simulink model "ps_25V_12kA_r"  (R2026b)
settings: Solver=ode23tb  StopTime=param.sim.simlength  FixedStep=param.glb_time.tc  MaxStep=param.glb_time.tc
values from neighbouring files (symbols this model uses):
  param = struct()    [init_model.m]
undefined symbols (not defined in the file or in its folder): magnitude
libraries: fl_lib x106, nesl_utility x71, afe_uvw_ctrl x5, ee_legacy_lib x5, discrete_time_low_pass_filter x2, three_windings_transformer x2, pi_ctrl x2, threephase_inductor_lib x1, dclink_for_two_levels x1, three_phase_pwm_modulator x1, three_phase_inverter_ideal_switch_based_model x1, three_phase_inverter_igbt_advanced_thermal_model x1
(part 3 of 5)

== system ps_25V_12kA_r/full_bridge_converter/phase_shift_full_bridge_ctrl/ui_ctrl ==
  i_pu_dab_input : Inport
  u_pu_dab_output : Inport  Port=2
  i_pu_dab_output_ref : Inport  Port=3
  i_ac_pu_1 : Inport  Port=4
  Trigger : TriggerPort  VariantControl=(inherit)  PortDimensions=1
  Goto Tag Visibility : GotoTagVisibility  GotoTag=idc_trafo_2
  Goto Tag Visibility1 : GotoTagVisibility  GotoTag=idc_trafo_1
  Goto Tag Visibility2 : GotoTagVisibility  GotoTag=idc_trafo_2_comp
  Goto Tag Visibility3 : GotoTagVisibility  GotoTag=idc_trafo_1_comp
  Goto Tag Visibility4 : GotoTagVisibility  GotoTag=i_pu_psfbc_output_ref
  Goto Tag Visibility5 : GotoTagVisibility  GotoTag=uout_pu_psfbc
  Goto Tag Visibility6 : GotoTagVisibility  GotoTag=i_ctrl_out_psfbc
  Goto Tag Visibility7 : GotoTagVisibility  GotoTag=i_pu_psfbc_output
  d1_m : Subsystem
  dc_trafo_current_measurements_and_compensation : Subsystem
  psfbc_ctrl : Subsystem
  scopes : Subsystem
  d1m : Outport
  phase_displacement : Outport  Port=2
  wires:
  i_pu_dab_input/1 -> psfbc_ctrl/1(i_pu_psfbc_output)
  u_pu_dab_output/1 -> psfbc_ctrl/2(u_pu_psfbc_output)
  i_pu_dab_output_ref/1 -> psfbc_ctrl/3(i_pu_psfbc_output_ref)
  psfbc_ctrl/1(phase_displacement) -> phase_displacement/1
  i_ac_pu_1/1 -> dc_trafo_current_measurements_and_compensation/1(i_ac_pu_1)
  d1_m/1(d1m) -> d1m/1

== system ps_25V_12kA_r/grid/grid_emulator/3ph_Dyg_ssc ==
  Electrical Reference1 : fl_lib/Electrical/Electrical Elements/Electrical Reference
  PS Terminator : fl_lib/Physical Signals/Sinks/PS Terminator
  PS Terminator1 : fl_lib/Physical Signals/Sinks/PS Terminator
  PS Terminator2 : fl_lib/Physical Signals/Sinks/PS Terminator
  configurable_trafo : SimscapeComponentBlock  Description=Configurable transformer: one or two three-phase primaries (star or delta), secondary three-phase (star or delta, any clock number) or single-phase (turns distribution ws) on a three-limb core. Component configurable_transformer.configurable_transformer (pwr-control/library, foundation/electrical_machines/+configurable_transformer).  SourceFile=configurable_transformer.configurable_transformer  ComponentPath=configurable_transformer.configurable_transformer  ComponentVariants="[\"configurable_transformer.configurable_transformer\"]"  ComponentVariantNames="[\"configurable_transformer\"]"  ClassName=configurable_transformer  SchemaVersion=1  primaries=configurable_transformer.n_primaries.one  conn1=configurable_transformer.connection.delta  conn2=configurable_transformer.connection.star  clock2=0  secondary=configurable_transformer.secondary_winding.star  clock3=param.grid.emu.trafo.pu.clock3  ws=[1, -1, 0]  Sr=param.grid.emu.trafo.pwr_nom A*V  V1=param.grid.emu.trafo.u1_nom V  V2=400 V  V3=param.grid.emu.trafo.u2_nom V  fr=param.grid.emu.trafo.f_nom Hz  r1=param.grid.emu.trafo.pu.r1  l1=param.grid.emu.trafo.pu.l1  r2=0.005  l2=0.030  r3=param.grid.emu.trafo.pu.r3  l3=param.grid.emu.trafo.pu.l3  lm=param.grid.emu.trafo.pu.lm  lm0=param.grid.emu.trafo.pu.lm0  rfe=param.grid.emu.trafo.pu.rfe  i1a_specify=off  i1a_priority=None  i1a=0 A  i1a_nominal_specify=off  i1a_nominal_value=1  i1a_nominal_unit=A  i1b_specify=off  i1b_priority=None  i1b=0 A  i1b_nominal_specify=off  i1b_nominal_value=1  i1b_nominal_unit=A  i1c_specify=off  i1c_priority=None  i1c=0 A  i1c_nominal_specify=off  i1c_nominal_value=1  i1c_nominal_unit=A  i2a_specify=off  i2a_priority=None  i2a=0 A  i2a_nominal_specify=off  i2a_nominal_value=1  i2a_nominal_unit=A  i2b_specify=off  i2b_priority=None  i2b=0 A  i2b_nominal_specify=off  i2b_nominal_value=1  i2b_nominal_unit=A  i2c_specify=off  i2c_priority=None  i2c=0 A  i2c_nominal_specify=off  i2c_nominal_value=1  i2c_nominal_unit=A  i3a_specify=off  i3a_priority=None  i3a=0 A  i3a_nominal_specify=off  i3a_nominal_value=1  i3a_nominal_unit=A  i3b_specify=off  i3b_priority=None  i3b=0 A  i3b_nominal_specify=off  i3b_nominal_value=1  i3b_nominal_unit=A  i3c_specify=off  i3c_priority=None  i3c=0 A  i3c_nominal_specify=off  i3c_nominal_value=1  i3c_nominal_unit=A  i3_specify=off  i3_priority=None  i3=0 A  i3_nominal_specify=off  i3_nominal_value=1  i3_nominal_unit=A
      settings: CopyFcn=simscape.sscblock.internal.componentBlockCallback(gcbh,'COPY')  PreCopyFcn=simscape.sscblock.internal.componentBlockCallback(gcbh,'PRECOPY')  PreDeleteFcn=simscape.sscblock.internal.componentBlockCallback(gcbh,'PREDELETE')
      mask Type: Configurable Transformer
  ua : PMIOPort  Side=Right
  ub : PMIOPort  Port=2  Side=Right
  uc : PMIOPort  Port=3  Side=Right
  Ua : PMIOPort  Port=4  Side=Left
  Ub : PMIOPort  Port=5  Side=Left
  Uc : PMIOPort  Port=6  Side=Left
  connections:
  Uc/RConn1 -- configurable_trafo/LConn3
  configurable_trafo/LConn2 -- Ub/RConn1
  configurable_trafo/RConn1 -- ua/RConn1
  configurable_trafo/LConn1 -- Ua/RConn1
  ub/RConn1 -- configurable_trafo/RConn2
  configurable_trafo/RConn3 -- uc/RConn1
  Electrical Reference1/LConn1 -- configurable_trafo/RConn4
  PS Terminator/LConn1 -- configurable_trafo/RConn5
  PS Terminator1/LConn1 -- configurable_trafo/RConn6
  configurable_trafo/RConn7 -- PS Terminator2/LConn1

== system ps_25V_12kA_r/grid/grid_emulator/threephase_vi_measures ==
  Bus Creator : BusCreator  Inputs=6
  Current Sensor : fl_lib/Electrical/Electrical Sensors/Current Sensor
  Current Sensor1 : fl_lib/Electrical/Electrical Sensors/Current Sensor
  Current Sensor2 : fl_lib/Electrical/Electrical Sensors/Current Sensor
  Electrical Reference1 : fl_lib/Electrical/Electrical Elements/Electrical Reference
  Voltage Sensor : fl_lib/Electrical/Electrical Sensors/Voltage Sensor
  Voltage Sensor1 : fl_lib/Electrical/Electrical Sensors/Voltage Sensor
  Voltage Sensor2 : fl_lib/Electrical/Electrical Sensors/Voltage Sensor
  i : Selector  InputPortWidth=6  IndexOptions=Index vector (dialog)  Indices=[4 5 6]  OutputSizes=1  RuntimeRangeChecks=off
  ia_grid : nesl_utility/PS-Simulink Converter  PhysicalDomain=network_engine_domain  SubClassName=ps_output  LeftPortType=input  RightPortType=output  PseudoPeriodic=off  Frequencies=[]  VectorFormat=1-D array  Unit=A  AffineConversion=off
  ib_grid : nesl_utility/PS-Simulink Converter  PhysicalDomain=network_engine_domain  SubClassName=ps_output  LeftPortType=input  RightPortType=output  PseudoPeriodic=off  Frequencies=[]  VectorFormat=1-D array  Unit=A  AffineConversion=off
  ic_grid : nesl_utility/PS-Simulink Converter  PhysicalDomain=network_engine_domain  SubClassName=ps_output  LeftPortType=input  RightPortType=output  PseudoPeriodic=off  Frequencies=[]  VectorFormat=1-D array  Unit=A  AffineConversion=off
  u : Selector  InputPortWidth=6  IndexOptions=Index vector (dialog)  Indices=[1 2 3]  OutputSizes=1  RuntimeRangeChecks=off
  ua_grid : nesl_utility/PS-Simulink Converter  PhysicalDomain=network_engine_domain  SubClassName=ps_output  LeftPortType=input  RightPortType=output  PseudoPeriodic=off  Frequencies=[]  VectorFormat=1-D array  Unit=V  AffineConversion=off
  ub_grid : nesl_utility/PS-Simulink Converter  PhysicalDomain=network_engine_domain  SubClassName=ps_output  LeftPortType=input  RightPortType=output  PseudoPeriodic=off  Frequencies=[]  VectorFormat=1-D array  Unit=V  AffineConversion=off
  uc_grid : nesl_utility/PS-Simulink Converter  PhysicalDomain=network_engine_domain  SubClassName=ps_output  LeftPortType=input  RightPortType=output  PseudoPeriodic=off  Frequencies=[]  VectorFormat=1-D array  Unit=V  AffineConversion=off
  Ua : PMIOPort  Side=Left
  ua : PMIOPort  Port=2  Side=Right
  Ub : PMIOPort  Port=3  Side=Left
  ub : PMIOPort  Port=4  Side=Right
  Uc : PMIOPort  Port=5  Side=Left
  uc : PMIOPort  Port=6  Side=Right
  tag scope: i_abc_line=global, u_abc_line=global
  wires:
  Bus Creator/1 -> i/1, u/1  "vi_data"
  ib_grid/1 -> Bus Creator/5  "ib"
  ia_grid/1 -> Bus Creator/4  "ia"
  ic_grid/1 -> Bus Creator/6  "ic"
  ua_grid/1 -> Bus Creator/1  "ua"
  ub_grid/1 -> Bus Creator/2  "ub"
  uc_grid/1 -> Bus Creator/3  "uc"
  i/1 -> [i_abc_line]
  u/1 -> [u_abc_line]
  connections:
  Current Sensor1/LConn1 -- Ub/RConn1 -- Voltage Sensor1/LConn1
  Electrical Reference1/LConn1 -- Voltage Sensor/RConn2 -- Voltage Sensor2/RConn2 -- Voltage Sensor1/RConn2
  Voltage Sensor/RConn1 -- ua_grid/LConn1
  Current Sensor/RConn2 -- ua/RConn1
  Voltage Sensor1/RConn1 -- ub_grid/LConn1
  Voltage Sensor2/LConn1 -- Current Sensor2/LConn1 -- Uc/RConn1
  Current Sensor/LConn1 -- Ua/RConn1 -- Voltage Sensor/LConn1
  Current Sensor1/RConn2 -- ub/RConn1
  Voltage Sensor2/RConn1 -- uc_grid/LConn1
  ib_grid/LConn1 -- Current Sensor1/RConn1
  ia_grid/LConn1 -- Current Sensor/RConn1
  ic_grid/LConn1 -- Current Sensor2/RConn1
  Current Sensor2/RConn2 -- uc/RConn1

== system ps_25V_12kA_r/afe_abc_mod1/AFE_control/afe_control/FRT-VDE4110 ==
  Constant4 : Constant  Value=0
  Mux : Mux
  Mux1 : Mux  Inputs=2
  enable : Step  Time=param.frt.data.settle_time  FinalValue=param.frt.data.enable_frt_1 + param.frt.data.enable_frt_2
  frt_detection_output : Scope  NumInputPorts=3
      settings: ActiveDisplayYMinimum=-0.12499999999999997  ActiveDisplayYMaximum=1.125
  frt_vde4110 : afe_uvw_ctrl/frt_vde4110  p=param.afe.uvw
  positive_reactive_current_reference : Subsystem
  reset : Step  Time=0.025  InitialValue=1  FinalValue=0
  tag scope: frt_active=scoped, i_grid_seq_ref=scoped, pwr_lim_enable=scoped
  wires:
  frt_vde4110/2 -> [frt_active], frt_detection_output/2  "frt_active"
  frt_vde4110/3 -> [pwr_lim_enable], frt_detection_output/3  "pwr_lim_enable"
  frt_vde4110/4 -> frt_detection_output/1  "frt_state"
  reset/1 -> frt_vde4110/4  "reset"
  enable/1 -> frt_vde4110/3  "enable"
  [v_grid_neg_eta_avg] -> Mux/4
  [v_grid_neg_xi_avg] -> Mux/3
  [v_grid_pos_eta_avg] -> Mux/2
  [v_grid_pos_xi_avg] -> Mux/1
  Mux/1 -> frt_vde4110/1
  positive_reactive_current_reference/1(i_react_pos_ref) -> [i_react_pos_ref]
  Constant4/1 -> [i_react_neg_ref]
  frt_vde4110/1 -> [i_grid_seq_ref]
  [i_react_neg_ref] -> Mux1/2
  [i_react_pos_ref] -> Mux1/1
  Mux1/1 -> frt_vde4110/2

== system ps_25V_12kA_r/afe_abc_mod1/AFE_control/afe_control/current_ctrl ==
  i_xi_ref : Inport
  Mux : Mux  Inputs=3
  current_ctrl_uvw : afe_uvw_ctrl/current_ctrl_uvw  p=param.afe.uvw
  isa_ref/isa : Scope  NumInputPorts=2
      settings: ActiveDisplayYMinimum=-3.5647345146351177  ActiveDisplayYMaximum=2.2290599372806974
  u_alpha_beta_gamma_out : Outport
  wires:
  i_xi_ref/1 -> current_ctrl_uvw/1  "is_pos_xi_ref"
  [i_stack_neg_xi_ref] -> Mux/2  "is_neg_xi_ref"
  [i_stack_pos_eta_ref] -> Mux/1  "is_pos_eta_ref"
  [i_stack_neg_eta_ref] -> Mux/3  "is_neg_eta_ref"
  [phase_grid_pll] -> current_ctrl_uvw/4
  [isd_abc_pu] -> current_ctrl_uvw/3
  current_ctrl_uvw/1 -> u_alpha_beta_gamma_out/1
  current_ctrl_uvw/2 -> isa_ref/isa/1
  current_ctrl_uvw/3 -> isa_ref/isa/2
  Mux/1 -> current_ctrl_uvw/2

== system ps_25V_12kA_r/afe_abc_mod1/AFE_control/afe_control/data_to_worspace_module_1 ==
  Bus Creator : BusCreator  Inputs=5
  dq_pll : Subsystem
  inner_current_tracking : Subsystem
  pwr_meter : Subsystem
  sequences_data : Subsystem
  m : Outport
  wires:
  Bus Creator/1 -> m/1
  sequences_data/1(m_seq) -> Bus Creator/1  "sequences_data"
  pwr_meter/1(m_pwr_meter) -> Bus Creator/2  "pwr_meter"
  inner_current_tracking/1(m_inner_current_tracking) -> Bus Creator/3  "m_inner_current_tracking"
  [local_time] -> Bus Creator/5  "local_time"
  dq_pll/1(dqPLLs) -> Bus Creator/4  "dq_pll"

== system ps_25V_12kA_r/afe_abc_mod1/AFE_control/afe_control/grid_current_sequences_and_reactive_pwr_ctrl ==
  ig_abc_pu : Inport
  Abs : Abs  SaturateOnIntegerOverflow=off
  Demux : Demux  Outputs=3
  Demux1 : Demux
  Saturation : Saturate  UpperLimit=2  LowerLimit=0.1
  Terminator : Terminator
  grid_current_sequences_q_ctrl : afe_uvw_ctrl/grid_current_sequences_q_ctrl  p=param.afe.uvw
  tag scope: i_grid_neg_eta_avg=scoped, i_grid_neg_xi_avg=scoped, i_grid_pos_eta_avg=scoped, i_grid_pos_xi_avg=scoped, i_stack_neg_eta_ref=scoped, i_stack_neg_xi_ref=scoped, i_stack_pos_eta_ref=scoped
  wires:
  [phase_grid_pll] -> grid_current_sequences_q_ctrl/2
  ig_abc_pu/1 -> grid_current_sequences_q_ctrl/1
  grid_current_sequences_q_ctrl/1 -> Demux/1
  Demux/1 -> [i_stack_pos_eta_ref]
  grid_current_sequences_q_ctrl/2 -> Demux1/1
  Demux1/1 -> [i_grid_pos_xi_avg]
  Demux1/2 -> [i_grid_pos_eta_avg]
  Demux1/3 -> [i_grid_neg_xi_avg]
  Demux1/4 -> [i_grid_neg_eta_avg]
  grid_current_sequences_q_ctrl/3 -> Terminator/1
  [i_grid_seq_ref] -> grid_current_sequences_q_ctrl/4
  Saturation/1 -> grid_current_sequences_q_ctrl/3
  [omega_grid_pll_pu] -> Abs/1
  Abs/1 -> Saturation/1
  Demux/2 -> [i_stack_neg_xi_ref]
  Demux/3 -> [i_stack_neg_eta_ref]

== system ps_25V_12kA_r/afe_abc_mod1/AFE_control/afe_control/grid_phase_acquisition ==
  grid_phase : Inport
  Quantizer : Quantizer  QuantizationInterval=param.meas.adc_quantization
  Unit Delay : UnitDelay  SampleTime=-1
  Zero-Order Hold : ZeroOrderHold  SampleTime=-1
  grid_phased : Outport
  wires:
  Zero-Order Hold/1 -> Quantizer/1
  Unit Delay/1 -> grid_phased/1
  grid_phase/1 -> Zero-Order Hold/1
  Quantizer/1 -> Unit Delay/1

== system ps_25V_12kA_r/afe_abc_mod1/AFE_control/afe_control/grid_voltage_phase_lock_loops ==
  ug_abc_pu : Inport
  Bus Creator2 : BusCreator  Inputs=2
  FHT-PLL performance : Scope  NumInputPorts=2
      settings: ActiveDisplayYMinimum=-1.32501220703125  ActiveDisplayYMaximum=1.30987548828125  DataLoggingVariableName=ScopeData8
  FHT-PLL_simulink : Subsystem
  tag scope: omega_grid_pll_pu=scoped, phase_grid_pll=scoped
  wires:
  FHT-PLL_simulink/1(gamma_grid_fht_pll) -> [phase_grid_pll]
  FHT-PLL_simulink/2(omega_grid_fht_pll) -> [omega_grid_pll_pu]
  ug_abc_pu/1 -> FHT-PLL performance/1, FHT-PLL_simulink/1(ug_abc_pu)
  Bus Creator2/1 -> FHT-PLL performance/2
  [omega_grid_pll_pu] -> Bus Creator2/2  "omega_grid_fht_pll"
  [phase_grid_pll] -> Bus Creator2/1  "phase_grid_fht_pll"

== system ps_25V_12kA_r/afe_abc_mod1/AFE_control/afe_control/grid_voltage_sequences ==
  Abs : Abs  SaturateOnIntegerOverflow=off
  Demux : Demux
  Demux1 : Demux  Outputs=2
  Saturation : Saturate  UpperLimit=2  LowerLimit=0.1
  Terminator : Terminator
  grid_voltage_sequences1 : afe_uvw_ctrl/grid_voltage_sequences  p=param.afe.uvw
  tag scope: ug_alpha_pu=scoped, ug_beta_pu=scoped, v_grid_neg_eta_avg=scoped, v_grid_neg_xi_avg=scoped, v_grid_pos_eta_avg=scoped, v_grid_pos_xi_avg=scoped
  wires:
  [ugd_abc_pu] -> grid_voltage_sequences1/1
  [phase_grid_pll] -> grid_voltage_sequences1/2
  Abs/1 -> Saturation/1
  [omega_grid_pll_pu] -> Abs/1
  Saturation/1 -> grid_voltage_sequences1/3
  grid_voltage_sequences1/1 -> Demux/1
  Demux/4 -> [v_grid_neg_eta_avg]
  Demux/3 -> [v_grid_neg_xi_avg]
  Demux/2 -> [v_grid_pos_eta_avg]
  Demux/1 -> [v_grid_pos_xi_avg]
  grid_voltage_sequences1/3 -> Demux1/1
  Demux1/1 -> [ug_alpha_pu]
  Demux1/2 -> [ug_beta_pu]
  grid_voltage_sequences1/2 -> Terminator/1

== system ps_25V_12kA_r/afe_abc_mod1/AFE_control/afe_control/ig afe quantizzation and one step delay ==
  ig_abc_pu : Inport
  Demux1 : Demux  Outputs=3
  Mux1 : Mux  Inputs=3
  ig afe quantizzation and one step delay : Subsystem
  igd_abc_pu : Outport
  wires:
  Demux1/1 -> ig afe quantizzation and one step delay/1(ig_u_pu)
  Demux1/2 -> ig afe quantizzation and one step delay/2(ig_v_pu)
  ig_abc_pu/1 -> Demux1/1
  Mux1/1 -> igd_abc_pu/1
  Demux1/3 -> ig afe quantizzation and one step delay/3(ig_w_pu)
  ig afe quantizzation and one step delay/2(igd_v_pu) -> Mux1/2
  ig afe quantizzation and one step delay/1(igd_u_pu) -> Mux1/1
  ig afe quantizzation and one step delay/3(igd_w_pu) -> Mux1/3

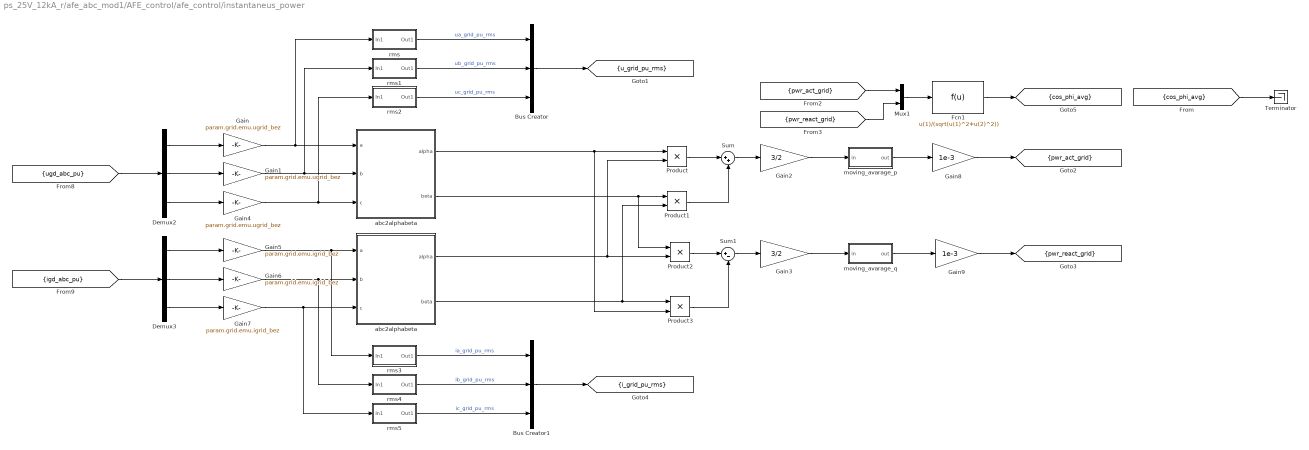
== system ps_25V_12kA_r/afe_abc_mod1/AFE_control/afe_control/instantaneus_power ==
  Bus Creator : BusCreator  Inputs=3
  Bus Creator1 : BusCreator  Inputs=3
  Demux2 : Demux  Outputs=3
  Demux3 : Demux  Outputs=3
  Fcn1 : Fcn  Expr=u(1)/(sqrt(u(1)^2+u(2)^2))
  Gain : Gain  Gain=param.grid.emu.ugrid_bez
  Gain1 : Gain  Gain=param.grid.emu.ugrid_bez
  Gain2 : Gain  Gain=3/2
  Gain3 : Gain  Gain=3/2
  Gain4 : Gain  Gain=param.grid.emu.ugrid_bez
  Gain5 : Gain  Gain=param.grid.emu.igrid_bez
  Gain6 : Gain  Gain=param.grid.emu.igrid_bez
  Gain7 : Gain  Gain=param.grid.emu.igrid_bez
  Gain8 : Gain  Gain=1e-3
  Gain9 : Gain  Gain=1e-3
  Mux1 : Mux  Inputs=2
  Product{,1..3} (4 alike) : Product  RndMeth=Zero
  Sum : Sum  Inputs=|++
  Sum1 : Sum  Inputs=|+-
  Terminator : Terminator
  abc2alphabeta : Subsystem
  "abc2alphabeta " : Subsystem
  moving_avarage_p : Subsystem
  moving_avarage_q : Subsystem
  rms : Subsystem
  rms1 : Subsystem
  rms2 : Subsystem
  rms3 : Subsystem
  rms4 : Subsystem
  rms5 : Subsystem
  tag scope: cos_phi_avg=scoped, i_grid_pu_rms=scoped, pwr_act_grid=scoped, pwr_react_grid=scoped, u_grid_pu_rms=scoped
  wires:
  abc2alphabeta/2("beta ") -> Product1/1, Product2/1
  "abc2alphabeta "/2("beta ") -> Product1/2, Product3/1
  abc2alphabeta/1("alpha ") -> Product3/2, Product/1
  "abc2alphabeta "/1("alpha ") -> Product2/2, Product/2
  Product/1 -> Sum/1
  Product1/1 -> Sum/2
  Product2/1 -> Sum1/1
  Product3/1 -> Sum1/2
  Sum1/1 -> Gain3/1
  Sum/1 -> Gain2/1
  Gain2/1 -> moving_avarage_p/1(in)
  Gain3/1 -> moving_avarage_q/1(in)
  [pwr_react_grid] -> Mux1/2
  Mux1/1 -> Fcn1/1
  Fcn1/1 -> [cos_phi_avg]
  [pwr_act_grid] -> Mux1/1
  rms/1(Out1) -> Bus Creator/1  "ua_grid_pu_rms"
  rms2/1(Out1) -> Bus Creator/3  "uc_grid_pu_rms"
  rms1/1(Out1) -> Bus Creator/2  "ub_grid_pu_rms"
  moving_avarage_p/1(out) -> Gain8/1
  moving_avarage_q/1(out) -> Gain9/1
  Demux2/1 -> Gain/1
  Demux2/2 -> Gain1/1
  Demux2/3 -> Gain4/1
  Demux3/1 -> Gain5/1
  Demux3/2 -> Gain6/1
  Demux3/3 -> Gain7/1
  Gain/1 -> rms/1(In1), abc2alphabeta/1(a)
  Gain1/1 -> rms1/1(In1), abc2alphabeta/2(b)
  Gain4/1 -> rms2/1(In1), abc2alphabeta/3(c)
  Gain5/1 -> rms3/1(In1), "abc2alphabeta "/1(a)
  Gain6/1 -> rms4/1(In1), "abc2alphabeta "/2(b)
  Gain7/1 -> rms5/1(In1), "abc2alphabeta "/3(c)
  Gain8/1 -> [pwr_act_grid]
  Gain9/1 -> [pwr_react_grid]
  [ugd_abc_pu] -> Demux2/1
  [igd_abc_pu] -> Demux3/1
  Bus Creator/1 -> [u_grid_pu_rms]
  rms4/1(Out1) -> Bus Creator1/2  "ib_grid_pu_rms"
  rms3/1(Out1) -> Bus Creator1/1  "ia_grid_pu_rms"
  rms5/1(Out1) -> Bus Creator1/3  "ic_grid_pu_rms"
  Bus Creator1/1 -> [i_grid_pu_rms]
  [cos_phi_avg] -> Terminator/1

== system ps_25V_12kA_r/afe_abc_mod1/AFE_control/afe_control/interesting scopes ==
  current_sequences_mod1 : Scope  NumInputPorts=4
      settings: ActiveDisplayYMinimum=-0.97178065031766891  ActiveDisplayYMaximum=1.9392475411295891  DataLoggingVariableName=ScopeData2
  i_grid_seq_ref : Scope
      settings: ActiveDisplayYMinimum=-1.1499999999999995  ActiveDisplayYMaximum=0.34999999999999981
  voltage_sequences_mod1 : Scope  NumInputPorts=4
      settings: ActiveDisplayYMinimum=-1.2405151816982258  ActiveDisplayYMaximum=1.2605257614333911
  wires:
  [v_grid_neg_eta_avg] -> voltage_sequences_mod1/4  "u_grid_neg_eta"
  [i_grid_neg_xi_avg] -> current_sequences_mod1/3  "i_grid_neg_xi"
  [v_grid_pos_eta_avg] -> voltage_sequences_mod1/2  "u_grid_pos_eta"
  [v_grid_neg_xi_avg] -> voltage_sequences_mod1/3  "u_grid_neg_xi"
  [i_grid_pos_xi_avg] -> current_sequences_mod1/1  "i_grid_pos_xi"
  [i_grid_neg_eta_avg] -> current_sequences_mod1/4  "i_grid_neg_eta"
  [v_grid_pos_xi_avg] -> voltage_sequences_mod1/1  "u_grid_pos_xi"
  [i_grid_pos_eta_avg] -> current_sequences_mod1/2  "i_grid_pos_eta"
  [i_grid_seq_ref] -> i_grid_seq_ref/1  "i_grid_seq_ref"

== system ps_25V_12kA_r/afe_abc_mod1/AFE_control/afe_control/is afe quantizzation and one step delay ==
  is_abc_pu : Inport
  Demux : Demux  Outputs=3
  Mux : Mux  Inputs=3
  is afe quantizzation and one step delay : Subsystem
  isd_abc_pu : Outport
  wires:
  is afe quantizzation and one step delay/2(isd_v_pu) -> Mux/2
  is_abc_pu/1 -> Demux/1
  is afe quantizzation and one step delay/3(isd_w_pu) -> Mux/3
  is afe quantizzation and one step delay/1(isd_u_pu) -> Mux/1
  Demux/1 -> is afe quantizzation and one step delay/1(is_u_pu)
  Mux/1 -> isd_abc_pu/1
  Demux/3 -> is afe quantizzation and one step delay/3(is_w_pu)
  Demux/2 -> is afe quantizzation and one step delay/2(is_v_pu)

== system ps_25V_12kA_r/afe_abc_mod1/AFE_control/afe_control/islanding_mode_detector ==
  gamma : Inport
  alpha : Inport  Port=2
  beta : Inport  Port=3
  Constant : Constant
  Mux : Mux  Inputs=2
  island_detection : Scope  NumInputPorts=3
      settings: ActiveDisplayYMinimum=-13.028939727220205  ActiveDisplayYMaximum=117.26045754498188  DataLoggingVariableName=ScopeData10
  islanding_detector : afe_uvw_ctrl/islanding_detector  p=param.afe.uvw
  wires:
  Mux/1 -> islanding_detector/1
  alpha/1 -> Mux/1  "u_grid_alpha"
  beta/1 -> Mux/2  "u_grid_beta"
  gamma/1 -> islanding_detector/2  "gamma_grid"
  [omega_grid_pll_pu] -> islanding_detector/3
  Constant/1 -> islanding_detector/4
  islanding_detector/1 -> island_detection/1
  islanding_detector/2 -> island_detection/2
  islanding_detector/3 -> island_detection/3

== system ps_25V_12kA_r/afe_abc_mod1/AFE_control/afe_control/phase_compensation_1 ==
  local_time : Inport
  master_time : Inport  Port=2
  Zero-Order Hold : ZeroOrderHold  SampleTime=-1
  Zero-Order Hold1 : ZeroOrderHold  SampleTime=-1
  alignment_eval_afe1 : Subsystem
  y : Outport
  wires:
  local_time/1 -> Zero-Order Hold/1
  master_time/1 -> Zero-Order Hold1/1
  alignment_eval_afe1/1(dp) -> y/1
  Zero-Order Hold/1 -> alignment_eval_afe1/1(local_time)
  Zero-Order Hold1/1 -> alignment_eval_afe1/2(master_time)

== system ps_25V_12kA_r/afe_abc_mod1/AFE_control/afe_control/space_vector ==
  uab_out : Inport
  Bus Creator : BusCreator  Inputs=3
  Bus Selector : BusSelector  OutputSignals=da,db,dc
  C Caller : CCaller  FunctionName=sv_pwm_cm_process_simulink  PortSpecificationStruct="%)30     .    B H   8    (     @         %    \"     8    !     0         %  0 \"0    $    _    07)G3F%M90  4&]R=$YA;64 4V-O<&4     26YD97@     5'EP90      4VEZ90      27-';&]B86P   X    P    !@    @    $          4    (     0    ,    !         !   P!O=70 #@   #     &    \"     0         !0    @    !     P    $         $  # &]U=  .    .     8    (    !          %    \"     $    &     0         0   ...(+3252 chars)"
  Constant : Constant  Value=param.glb_time.ts_afe
  Constant1 : Constant
  Data Type Conversion1 : DataTypeConversion  OutDataTypeStr=double  SaturateOnIntegerOverflow=off  RndMeth=Floor
  Data Type Conversion{4,15..16,18} (4 alike) : DataTypeConversion  OutDataTypeStr=single  SaturateOnIntegerOverflow=off  RndMeth=Floor
  Data Type Conversion17 : DataTypeConversion  OutDataTypeStr=uint32  SaturateOnIntegerOverflow=off  RndMeth=Floor
  Data Type Conversion2 : DataTypeConversion  OutDataTypeStr=double  SaturateOnIntegerOverflow=off  RndMeth=Floor
  Data Type Conversion3 : DataTypeConversion  OutDataTypeStr=double  SaturateOnIntegerOverflow=off  RndMeth=Floor
  Demux : Demux  Outputs=3
  Gain1 : Gain  Gain=sqrt(3)/2
  Gain2 : Gain  Gain=sqrt(3)/2
  Gain3 : Gain  Gain=param.afe.ref.u_cm_comp_mod1
  duvw : Outport
  wires:
  Data Type Conversion15/1 -> C Caller/2
  Bus Selector/2 -> Data Type Conversion2/1  "<db>"
  Data Type Conversion18/1 -> C Caller/1
  C Caller/1 -> Bus Selector/1
  Bus Creator/1 -> duvw/1
  Data Type Conversion1/1 -> Bus Creator/1  "du(k)"
  Demux/2 -> Gain2/1
  Bus Selector/3 -> Data Type Conversion3/1  "<dc>"
  Demux/1 -> Gain1/1
  Data Type Conversion2/1 -> Bus Creator/2  "dv(k)"
  Gain2/1 -> Data Type Conversion15/1
  Bus Selector/1 -> Data Type Conversion1/1  "<da>"
  Gain1/1 -> Data Type Conversion18/1
  Data Type Conversion3/1 -> Bus Creator/3  "dw(k)"
  Constant/1 -> Data Type Conversion16/1
  uab_out/1 -> Demux/1
  Constant1/1 -> Data Type Conversion17/1
  Data Type Conversion16/1 -> C Caller/4
  Data Type Conversion17/1 -> C Caller/5
  Demux/3 -> Gain3/1
  Gain3/1 -> Data Type Conversion4/1
  Data Type Conversion4/1 -> C Caller/3

== system ps_25V_12kA_r/afe_abc_mod1/AFE_control/afe_control/udc_acquisition ==
  udc_pu : Inport
  Quantizer : Quantizer  QuantizationInterval=param.meas.adc_quantization
  Unit Delay : UnitDelay  SampleTime=-1
  Zero-Order Hold : ZeroOrderHold  SampleTime=-1
  udcd_pu : Outport
  wires:
  Quantizer/1 -> Unit Delay/1
  udc_pu/1 -> Zero-Order Hold/1
  Unit Delay/1 -> udcd_pu/1
  Zero-Order Hold/1 -> Quantizer/1

== system ps_25V_12kA_r/afe_abc_mod1/AFE_control/afe_control/udc_ctrl ==
  udc_pu : Inport
  1/Ti : Gain  Gain=param.afe.ctrl.kp_udc_ctrl  SaturateOnIntegerOverflow=on  OutDataTypeStr=Inherit: Same as input  ParamDataTypeStr=Inherit: Same as input
  Constant : Constant  Value=0
  Gain : Gain  Gain=-1
  Saturation : Saturate  UpperLimit=param.afe.ctrl.ixi_pos_ref_lim  LowerLimit=-param.afe.ctrl.ixi_pos_ref_lim
  Sum1 : Sum  Inputs=+++  SaturateOnIntegerOverflow=on
  Sum2 : Sum  Inputs=-+  SaturateOnIntegerOverflow=on
  Sum3 : Sum  Inputs=-+  SaturateOnIntegerOverflow=on
  Switch : Switch  Criteria=u2 > Threshold  SaturateOnIntegerOverflow=off  InputSameDT=off
  To Workspace1 : ToWorkspace  VariableName=udc_pu_sim_mod1  SampleTime=-1
      settings: MaxDataPoints=param.glb_time.Ns_afe
  To Workspace3 : ToWorkspace  VariableName=udc_pu_ref_sim_mod1  SampleTime=-1
      settings: MaxDataPoints=param.glb_time.Ns_afe
  Unit Delay4 : UnitDelay  SampleTime=-1
  discrete-time-low-pass-filter1 : discrete_time_low_pass_filter/discrete-time-low-pass-filter  tau=20e-3  ts=param.glb_time.ts_afe
  kp : Gain  Gain=param.afe.ctrl.ki_udc_ctrl*param.glb_time.ts_afe  SaturateOnIntegerOverflow=on  OutDataTypeStr=Inherit: Same as input  ParamDataTypeStr=Inherit: Same as input
  udc_norm_ref : Step  Time=1e-3  FinalValue=param.afe.ctrl.udc_norm_ref
  udc_tracking : Scope  NumInputPorts=3
      settings: ActiveDisplayYMinimum=-2.0004150390624997  ActiveDisplayYMaximum=1.5037353515624998  DataLoggingVariableName=ScopeData8
  i_xi_ref : Outport
  wires:
  1/Ti/1 -> Sum1/1, Sum3/1
  kp/1 -> Sum1/2
  Sum3/1 -> Unit Delay4/1
  Unit Delay4/1 -> Sum1/3
  udc_norm_ref/1 -> discrete-time-low-pass-filter1/1
  udc_pu/1 -> Sum2/1, To Workspace1/1, udc_tracking/2  "udc_pu"
  Sum2/1 -> kp/1, 1/Ti/1
  Sum1/1 -> Saturation/1
  [pwr_lim_enable] -> Switch/2
  Saturation/1 -> Switch/3
  Switch/1 -> Sum3/2, Gain/1
  Constant/1 -> Switch/1
  Gain/1 -> udc_tracking/3, i_xi_ref/1  "i_xi_ref"
  discrete-time-low-pass-filter1/1 -> To Workspace3/1, udc_tracking/1, Sum2/2  "udc_pu_ref"

== system ps_25V_12kA_r/afe_abc_mod1/AFE_control/afe_control/ug afe quantizzation and one step delay ==
  ug_abc_pu : Inport
  Demux : Demux  Outputs=3
  Mux : Mux  Inputs=3
  ug afe quantizzation and one step delay : Subsystem
  ugd_abc_pu : Outport
  wires:
  ug afe quantizzation and one step delay/2(ugd_v_pu) -> Mux/2
  Demux/2 -> ug afe quantizzation and one step delay/2(ug_v_pu)
  Demux/3 -> ug afe quantizzation and one step delay/3(ug_w_pu)
  ug afe quantizzation and one step delay/1(ugd_u_pu) -> Mux/1
  Demux/1 -> ug afe quantizzation and one step delay/1(ug_u_pu)
  ug_abc_pu/1 -> Demux/1
  ug afe quantizzation and one step delay/3(ugd_w_pu) -> Mux/3
  Mux/1 -> ugd_abc_pu/1

== system ps_25V_12kA_r/afe_abc_mod1/afe/sv_pwm/modulator1 ==
  u : Inport
  v : Inport  Port=2
  w : Inport  Port=3
  phase : Inport  Port=4
  Bus Creator : BusCreator  Inputs=3
  Three phase two level PWM generator with global TRGO : three_phase_pwm_modulator/Three phase two level PWM generator with global TRGO  f=param.glb_time.fPWM_AFE  m_up=0.98  m_low=0.02  dead_time=param.glb_time.dead_time_AFE  pos_cmd_gate=15  neg_cmd_gate=-10  polarity=1  tc=param.glb_time.tc  double_sampling=1
      link override gate commands/Bus Selector: OutputSignals=du(t)
      link override gate commands/Bus Selector1: OutputSignals=dv(t)
      link override gate commands/Bus Selector2: OutputSignals=dw(t)
  gate_cmds : Outport
  tag scope: TRGO_afe_module_1=global
  wires:
  [time_afe_module_1] -> Three phase two level PWM generator with global TRGO/1
  Bus Creator/1 -> Three phase two level PWM generator with global TRGO/3
  Three phase two level PWM generator with global TRGO/1 -> [TRGO_afe_module_1]
  u/1 -> Bus Creator/1
  v/1 -> Bus Creator/2
  w/1 -> Bus Creator/3
  phase/1 -> Three phase two level PWM generator with global TRGO/2
  Three phase two level PWM generator with global TRGO/2 -> gate_cmds/1

== system ps_25V_12kA_r/full_bridge_converter/full_bridge_converter_with_iso/full_bridge/full-bridge_ideal_switch_based ==
  gate_commands : Inport
  full-bridge ideal switch based : full_bridge_ideal_switch/full-bridge ideal switch based  Rds_on=param.psfbc.ideal_switch.Rds_on  Vdon_diode=param.psfbc.ideal_switch.Vdon_diode  Rdon_diode=param.psfbc.ideal_switch.Rdon_diode  Csnubber=param.psfbc.ideal_switch.Csnubber  Rsnubber=param.psfbc.ideal_switch.Rsnubber  Vth=param.psfbc.ideal_switch.Vth
  udc(+) : PMIOPort  Side=Left
  uac(+) : PMIOPort  Port=2  Side=Right
  udc(-) : PMIOPort  Port=3  Side=Left
  uac(-) : PMIOPort  Port=4  Side=Right
  tag scope: full_bridge_ideal_switch_data=global
  wires:
  full-bridge ideal switch based/1 -> [full_bridge_ideal_switch_data]
  gate_commands/1 -> full-bridge ideal switch based/1
  connections:
  uac(-)/RConn1 -- full-bridge ideal switch based/RConn2
  udc(-)/RConn1 -- full-bridge ideal switch based/LConn2
  full-bridge ideal switch based/RConn1 -- uac(+)/RConn1
  udc(+)/RConn1 -- full-bridge ideal switch based/LConn1

== system ps_25V_12kA_r/full_bridge_converter/full_bridge_converter_with_iso/full_bridge/full-bridge_mosfet_based_ with_thermal_model_zvs ==
  gate_commands : Inport
  full-bridge_mosfet_based_ with_thermal_model_zvs : full_bridge_mosfet_based_with_thermal_model_zvs/full-bridge_mosfet_based_ with_thermal_model_zvs  mass_heatsink_m=param.thermal.heatsink.no_weight  specific_heat_m=param.thermal.heatsink.cp  rth_mosfet_HA_m=param.thermal.heatsink.Rth_mosfet_HA  rth_mosfet_JH_m=param.psfbc.mosfet.Rth_mosfet_JH  Rds_on_m=param.psfbc.mosfet.Rds_on  Vth_m=param.psfbc.mosfet.Vth  Eon_m=param.psfbc.mosfet.Eon  Eoff_m=param.psfbc.mosfet.Eoff  Voff_sw_loss_m=param.psfbc.mosfet.Voff_sw_losses  Ion_sw_loss_m=param.psfbc.mosfet.Ion_sw_losses  Vdon_diode_m=param.psfbc.mosfet.Vdon_diode  Rdon_diode_m=param.psfbc.mosfet.Rds_on  JunctionTermalMass_m=param.psfbc.mosfet.JunctionTermalMass  Tambient_m=param.thermal.heatsink.Tambient  DThs_init_m=param.thermal.heatsink.DThs_init  Csnubber_m=param.psfbc.mosfet.Csnubber_zvs  Rsnubber_m=param.psfbc.mosfet.Rsnubber_zvs
  udc(+) : PMIOPort  Side=Left
  uac(+) : PMIOPort  Port=2  Side=Right
  uac(-) : PMIOPort  Port=3  Side=Right
  udc(-) : PMIOPort  Port=4  Side=Left
  tag scope: full_bridge_mosfet_data=global
  wires:
  gate_commands/1 -> full-bridge_mosfet_based_ with_thermal_model_zvs/1
  full-bridge_mosfet_based_ with_thermal_model_zvs/1 -> [full_bridge_mosfet_data]
  connections:
  full-bridge_mosfet_based_ with_thermal_model_zvs/RConn2 -- uac(-)/RConn1
  full-bridge_mosfet_based_ with_thermal_model_zvs/LConn1 -- udc(+)/RConn1
  full-bridge_mosfet_based_ with_thermal_model_zvs/RConn1 -- uac(+)/RConn1
  full-bridge_mosfet_based_ with_thermal_model_zvs/LConn2 -- udc(-)/RConn1

== system ps_25V_12kA_r/full_bridge_converter/full_bridge_converter_with_iso/full_bridge/full_bridge_igbt_adv_thermal_model ==
  gate_commands : Inport
  data_reference : Subsystem
  full_bridge_igbt_adv_thermal_model : full_bridge_igbt_based_with_advanced_thermal_model/full_bridge_igbt_adv_thermal_model  mass_heatsink_m=param.thermal.heatsink.no_weight  specific_heat_m=param.thermal.heatsink.cp  rth_switch_HA_m=param.thermal.heatsink.Rth_switch_HA  rth_switch_JH_m=param.psfbc.igbt.Rth_switch_JH  rth_diode_HA_m=param.thermal.heatsink.Rth_diode_HA  rth_diode_JH_m=param.psfbc.igbt.Rth_diode_JH  Rce_on_m=param.psfbc.igbt.Rce_on  Vce_sat_m=param.psfbc.igbt.Vce_sat  Vth_m=param.psfbc.igbt.Vth  Eon_m=param.psfbc.igbt.Eon  Eoff_m=param.psfbc.igbt.Eoff  Erec_m=param.psfbc.igbt.Erec  Irr_m=param.psfbc.igbt.Irr  Voff_sw_loss_m=param.psfbc.igbt.Voff_sw_losses  Ion_sw_loss_m=param.psfbc.igbt.Ion_sw_losses  Vdon_diode_m=param.psfbc.igbt.Vdon_diode  Rdon_diode_m=param.psfbc.igbt.Rdon_diode  Csnubber_m=param.psfbc.igbt.Csnubber  Rsnubber_m=param.psfbc.igbt.Rsnubber  JunctionTermalMass_m=param.psfbc.igbt.JunctionTermalMass  Tambient_m=param.thermal.heatsink.Tambient  DThs_init_m=param.thermal.heatsink.DThs_init  Lstray_module_m=param.psfbc.igbt.Lstray_module  Cies_m=param.psfbc.igbt.Cies  tc_m=param.glb_time.tc
  udc(+) : PMIOPort  Side=Left
  uac(+) : PMIOPort  Port=2  Side=Right
  udc(-) : PMIOPort  Port=3  Side=Left
  uac(-) : PMIOPort  Port=4  Side=Right
  wires:
  full_bridge_igbt_adv_thermal_model/1 -> data_reference/1(m)
  gate_commands/1 -> full_bridge_igbt_adv_thermal_model/1
  connections:
  full_bridge_igbt_adv_thermal_model/LConn2 -- udc(-)/RConn1
  full_bridge_igbt_adv_thermal_model/RConn2 -- uac(-)/RConn1
  full_bridge_igbt_adv_thermal_model/LConn1 -- udc(+)/RConn1
  full_bridge_igbt_adv_thermal_model/RConn1 -- uac(+)/RConn1

== system ps_25V_12kA_r/full_bridge_converter/full_bridge_converter_with_iso/trafo_rectifier/rectifiers ==
  CFu_dc2 : fl_lib/Electrical/Electrical Elements/Capacitor  c=param.psfbc.hw.Cdc_dc2 F  r=param.psfbc.hw.RCdc_dc2 Ohm  g=0 1/Ohm  i_specify=off  i_priority=None  i=0 A  i_nominal_specify=off  i_nominal_value=1  i_nominal_unit=A  v_specify=off  v_priority=None  v=0 V  v_nominal_specify=off  v_nominal_value=1  v_nominal_unit=V  vc_specify=off  vc_priority=High  vc=0 V  vc_nominal_specify=off  vc_nominal_value=1  vc_nominal_unit=V
  Current Sensor1 : fl_lib/Electrical/Electrical Sensors/Current Sensor
  Current Sensor3 : fl_lib/Electrical/Electrical Sensors/Current Sensor
  Current Sensor5 : fl_lib/Electrical/Electrical Sensors/Current Sensor
  PS-Simulink Converter2 : nesl_utility/PS-Simulink Converter  PhysicalDomain=network_engine_domain  SubClassName=ps_output  LeftPortType=input  RightPortType=output  PseudoPeriodic=off  Frequencies=[]  VectorFormat=1-D array  Unit=A  AffineConversion=on
  Voltage Sensor1 : fl_lib/Electrical/Electrical Sensors/Voltage Sensor
  idc1 : nesl_utility/PS-Simulink Converter  PhysicalDomain=network_engine_domain  SubClassName=ps_output  LeftPortType=input  RightPortType=output  PseudoPeriodic=off  Frequencies=[]  VectorFormat=1-D array  Unit=A  AffineConversion=off
  idc2 : nesl_utility/PS-Simulink Converter  PhysicalDomain=network_engine_domain  SubClassName=ps_output  LeftPortType=input  RightPortType=output  PseudoPeriodic=off  Frequencies=[]  VectorFormat=1-D array  Unit=A  AffineConversion=off
  rectifier : Subsystem
  udc2 : nesl_utility/PS-Simulink Converter  PhysicalDomain=network_engine_domain  SubClassName=ps_output  LeftPortType=input  RightPortType=output  PseudoPeriodic=off  Frequencies=[]  VectorFormat=1-D array  Unit=V  AffineConversion=off
  uac_2(+) : PMIOPort  Side=Left
  uac_3(-) : PMIOPort  Port=2  Side=Left
  un(-) : PMIOPort  Port=3  Side=Left
  udc_load(+) : PMIOPort  Port=4  Side=Right
  udc_load(-) : PMIOPort  Port=5  Side=Right
  uac_4(+) : PMIOPort  Port=6  Side=Left
  uac_5(-) : PMIOPort  Port=7  Side=Left
  tag scope: CFu_dc2_current=global, LFu_dc2_current=global, diode_rectifiers=global, psfbc_current_output=global, psfbc_voltage_output=global
  wires:
  PS-Simulink Converter2/1 -> [CFu_dc2_current]  "CFu_dc2_current"
  udc2/1 -> [psfbc_voltage_output]  "psfbc_voltage_output"
  idc2/1 -> [psfbc_current_output]  "psfbc_current_output"
  idc1/1 -> [LFu_dc2_current]  "LFu_dc2_current"
  rectifier/1(m) -> [diode_rectifiers]
  connections:
  CFu_dc2/LConn1 -- Current Sensor5/RConn2 -- Current Sensor3/LConn1 -- Voltage Sensor1/LConn1
  idc1/LConn1 -- Current Sensor5/RConn1
  Current Sensor3/RConn2 -- udc_load(+)/RConn1
  Current Sensor1/RConn2 -- rectifier/RConn2 -- Voltage Sensor1/RConn2 -- udc_load(-)/RConn1
  CFu_dc2/RConn1 -- Current Sensor1/LConn1
  Voltage Sensor1/RConn1 -- udc2/LConn1
  idc2/LConn1 -- Current Sensor3/RConn1
  PS-Simulink Converter2/LConn1 -- Current Sensor1/RConn1
  rectifier/LConn1 -- uac_2(+)/RConn1
  uac_3(-)/RConn1 -- rectifier/LConn2
  rectifier/LConn4 -- uac_5(-)/RConn1
  rectifier/LConn3 -- uac_4(+)/RConn1
  Current Sensor5/LConn1 -- rectifier/RConn1
  un(-)/RConn1 -- rectifier/LConn5

== system ps_25V_12kA_r/full_bridge_converter/full_bridge_converter_with_iso/trafo_rectifier/transformers ==
  Current Sensor1 : fl_lib/Electrical/Electrical Sensors/Current Sensor
  Voltage Sensor1 : fl_lib/Electrical/Electrical Sensors/Voltage Sensor
  i1_psfbc_transformer : nesl_utility/PS-Simulink Converter  PhysicalDomain=network_engine_domain  SubClassName=ps_output  LeftPortType=input  RightPortType=output  PseudoPeriodic=off  Frequencies=[]  VectorFormat=1-D array  Unit=A  AffineConversion=off
  trafo_1 : Subsystem
  trafo_2 : Subsystem  Commented=on
  u1_psfbc_transformer : nesl_utility/PS-Simulink Converter  PhysicalDomain=network_engine_domain  SubClassName=ps_output  LeftPortType=input  RightPortType=output  PseudoPeriodic=off  Frequencies=[]  VectorFormat=1-D array  Unit=V  AffineConversion=on
  uac_1(+) : PMIOPort  Side=Left
  uac_1(-) : PMIOPort  Port=2  Side=Left
  uac_2(+) : PMIOPort  Port=3  Side=Right
  uac_3(-) : PMIOPort  Port=4  Side=Right
  un(-) : PMIOPort  Port=5  Side=Right
  uac_4(+) : PMIOPort  Port=6  Side=Right
  uac_5(-) : PMIOPort  Port=7  Side=Right
  tag scope: i1_psfbc_transformer=global, u1_psfbc_transformer=global
  wires:
  u1_psfbc_transformer/1 -> [u1_psfbc_transformer]
  i1_psfbc_transformer/1 -> [i1_psfbc_transformer]
  connections:
  trafo_2/LConn1 -- trafo_1/LConn1 -- Current Sensor1/RConn2
  uac_1(-)/RConn1 -- Voltage Sensor1/RConn2 -- trafo_2/LConn2 -- trafo_1/LConn2
  trafo_1/RConn1 -- uac_2(+)/RConn1
  trafo_1/RConn2 -- uac_3(-)/RConn1
  trafo_1/RConn3 -- trafo_2/RConn3 -- un(-)/RConn1
  uac_4(+)/RConn1 -- trafo_2/RConn1
  trafo_2/RConn2 -- uac_5(-)/RConn1
  Voltage Sensor1/LConn1 -- Current Sensor1/LConn1 -- uac_1(+)/RConn1
  Voltage Sensor1/RConn1 -- u1_psfbc_transformer/LConn1
  Current Sensor1/RConn1 -- i1_psfbc_transformer/LConn1

== system ps_25V_12kA_r/full_bridge_converter/phase_shift_full_bridge_ctrl/ui_ctrl/d1_m ==
  Constant : Constant  Value=0.5
  Sum : Sum  Inputs=|++
  d1m : Outport
  wires:
  Constant/1 -> Sum/1
  Sum/1 -> d1m/1

== system ps_25V_12kA_r/full_bridge_converter/phase_shift_full_bridge_ctrl/ui_ctrl/dc_trafo_current_measurements_and_compensation ==
  i_ac_pu_1 : Inport
  Constant : Constant  Value=0
  Gain : Gain  Gain=1/2
  Gain3 : Gain
  Quantizer1 : Quantizer  QuantizationInterval=param.meas.adc12_quantization
  Sum1 : Sum  Inputs=|++
  To Workspace3 : ToWorkspace  VariableName=idc_trafo_1  SampleTime=-1
      settings: MaxDataPoints=param.glb_time.Ns_dab
  To Workspace4 : ToWorkspace  VariableName=i_ac_pu_1_sim  SampleTime=-1
      settings: MaxDataPoints=param.glb_time.Ns_dab
  Unit Delay2 : UnitDelay  SampleTime=-1
  Unit Delay3 : UnitDelay  SampleTime=-1
  Zero-Order Hold : ZeroOrderHold  SampleTime=-1
  discrete-time-low-pass-filter1 : discrete_time_low_pass_filter/discrete-time-low-pass-filter  tau=param.psfbc.ctrl.tau_idc_trafo  ts=param.glb_time.ts_dab
  i_ac_pu_1/2 : Scope  NumInputPorts=3
      settings: ActiveDisplayYMinimum=-1.2874755859375  ActiveDisplayYMaximum=3.7943115234375  DataLoggingVariableName=ScopeData14
  pi_ctrl_idc_trafo_1 : pi_ctrl/pi_ctrl  kp=param.psfbc.ctrl.kp_idc_trafo  ki=param.psfbc.ctrl.ki_idc_trafo  ts=param.glb_time.ts_dab  lim_up=param.psfbc.ctrl.lim_idc_trafo  lim_down=-param.psfbc.ctrl.lim_idc_trafo
  tag scope: idc_trafo_1=scoped, idc_trafo_1_comp=scoped
  wires:
  i_ac_pu_1/1 -> Zero-Order Hold/1
  Quantizer1/1 -> Unit Delay2/1
  Unit Delay2/1 -> Sum1/1, Unit Delay3/1, i_ac_pu_1/2/1, To Workspace4/1  "i_ac_pu_1"
  Zero-Order Hold/1 -> Quantizer1/1
  Unit Delay3/1 -> Sum1/2  "i_ac_pu_1"
  Sum1/1 -> Gain/1
  Gain/1 -> discrete-time-low-pass-filter1/1  "idc_trafo_1"
  discrete-time-low-pass-filter1/1 -> To Workspace3/1, [idc_trafo_1], i_ac_pu_1/2/3  "idc_trafo_1"
  [idc_trafo_1] -> pi_ctrl_idc_trafo_1/2
  Constant/1 -> pi_ctrl_idc_trafo_1/3, pi_ctrl_idc_trafo_1/1
  pi_ctrl_idc_trafo_1/1 -> Gain3/1
  Gain3/1 -> [idc_trafo_1_comp]  "idc_trafo_1_comp"
  [idc_trafo_1_comp] -> i_ac_pu_1/2/2  "idc_trafo_1_comp"

== system ps_25V_12kA_r/full_bridge_converter/phase_shift_full_bridge_ctrl/ui_ctrl/psfbc_ctrl ==
  i_pu_psfbc_output : Inport
  u_pu_psfbc_output : Inport  Port=2
  i_pu_psfbc_output_ref : Inport  Port=3
  Quantizer1 : Quantizer  QuantizationInterval=param.meas.adc12_quantization
  Quantizer2 : Quantizer  QuantizationInterval=param.meas.adc12_quantization
  Unit Delay2 : UnitDelay  SampleTime=-1
  Unit Delay3 : UnitDelay  SampleTime=-1
  current control : Subsystem
  phase_displacement : Outport
  tag scope: i_ctrl_out_psfbc=scoped, i_pu_psfbc_output=scoped, i_pu_psfbc_output_ref=scoped, uout_pu_psfbc=scoped
  wires:
  i_pu_psfbc_output_ref/1 -> [i_pu_psfbc_output_ref], current control/1(iout_ref)  "iout_ref"
  i_pu_psfbc_output/1 -> Quantizer2/1
  current control/1(i_ctrl_out) -> phase_displacement/1, [i_ctrl_out_psfbc]
  Unit Delay3/1 -> current control/2(iout), [i_pu_psfbc_output]
  Unit Delay2/1 -> [uout_pu_psfbc]
  u_pu_psfbc_output/1 -> Quantizer1/1
  Quantizer1/1 -> Unit Delay2/1
  Quantizer2/1 -> Unit Delay3/1

== system ps_25V_12kA_r/full_bridge_converter/phase_shift_full_bridge_ctrl/ui_ctrl/scopes ==
  Bus Creator : BusCreator  Inputs=2
  Bus Creator1 : BusCreator  Inputs=2
  From7 : From  Commented=on  GotoTag=uout_ref_pu_psfbc
  psfbc-tracking : Scope  NumInputPorts=2
      settings: ActiveDisplayYMinimum=-0.7264395439314022  ActiveDisplayYMaximum=2.2614067014075516  DataLoggingVariableName=ScopeData7
  u_ctrl_out_psfbc/i_ctrl_out_psfbc : Scope  NumInputPorts=2
      settings: ActiveDisplayYMinimum=-1.2812486231311795  ActiveDisplayYMaximum=1.531237608180616
  wires:
  Bus Creator1/1 -> psfbc-tracking/2
  Bus Creator/1 -> psfbc-tracking/1
  [i_ctrl_out_psfbc] -> u_ctrl_out_psfbc/i_ctrl_out_psfbc/2  "i_ctrl_out_psfbc"
  [i_pu_psfbc_output] -> Bus Creator1/2  "i_in_pu_psfbc"
  From7/1 -> Bus Creator/1  "uout_ref_pu_psfbc"
  [i_pu_psfbc_output_ref] -> u_ctrl_out_psfbc/i_ctrl_out_psfbc/1  "u_ctrl_out_psfbc"
  [i_pu_psfbc_output_ref] -> Bus Creator1/1  "u_ctrl_out_psfbc"
  [uout_pu_psfbc] -> Bus Creator/2  "uout_pu_psfbc"

== system ps_25V_12kA_r/afe_abc_mod1/AFE_control/afe_control/FRT-VDE4110/positive_reactive_current_reference ==
  Step : Step  Time=param.afe.ref.time_i_react_pos_ref_1  InitialValue=param.afe.ref.i_react_pos_ref_1  FinalValue=param.afe.ref.i_react_pos_ref_2
  Step1 : Step  Time=param.afe.ref.time_i_react_pos_ref_2  FinalValue=param.afe.ref.i_react_pos_ref_3-param.afe.ref.i_react_pos_ref_2
  Sum7 : Sum  Inputs=|++
  i_react_pos_ref : Outport
  wires:
  Sum7/1 -> i_react_pos_ref/1
  Step1/1 -> Sum7/2
  Step/1 -> Sum7/1

== system ps_25V_12kA_r/afe_abc_mod1/AFE_control/afe_control/data_to_worspace_module_1/dq_pll ==
  Bus Creator1 : BusCreator  Inputs=8
  dqPLLs : Outport
  wires:
  [phase_grid_fht_simulink_pll] -> Bus Creator1/5  "phase_grid_fht_simulink_pll"
  [omega_grid_fht_simulink_pll] -> Bus Creator1/6  "omega_grid_fht_simulink_pll"
  [omega_grid_fhtsr_dqpll] -> Bus Creator1/8  "omega_grid_fhtsr_dqpll"
  [phase_grid_fhtsr_dqpll] -> Bus Creator1/7  "phase_grid_fhtsr_dqpll"
  [omega_grid_dqpll_ccaller] -> Bus Creator1/4  "omega_grid_dqpll_ccaller"
  [phase_grid_dqpll_ccaller] -> Bus Creator1/3  "phase_grid_dqpll_ccaller"
  [omega_grid_pu_dqpll] -> Bus Creator1/2  "omega_grid_pu_dqpll"
  [phase_grid_dqpll] -> Bus Creator1/1  "phase_grid_dqpll"
  Bus Creator1/1 -> dqPLLs/1

== system ps_25V_12kA_r/afe_abc_mod1/AFE_control/afe_control/data_to_worspace_module_1/inner_current_tracking ==
  Bus Creator1 : BusCreator  Inputs=11
  m_inner_current_tracking : Outport
  wires:
  [iz_pu] -> Bus Creator1/10  "iz_pu"
  [id_eta_pu] -> Bus Creator1/2  "i_eta_pu"
  [isc] -> Bus Creator1/8  "isc_pu"
  [isa_ref] -> Bus Creator1/3  "isa_pu_ref"
  [isa] -> Bus Creator1/4  "isa_pu"
  [id_xi_pu] -> Bus Creator1/1  "i_xi_pu"
  [iz_pu_ref] -> Bus Creator1/9  "iz_pu_ref"
  [isb] -> Bus Creator1/6  "isb_pu"
  [isb_ref] -> Bus Creator1/5  "isb_pu_ref"
  [iz_ctrl_out] -> Bus Creator1/11  "iz_ctrl_out"
  [isc_ref] -> Bus Creator1/7  "isc_pu_ref"
  Bus Creator1/1 -> m_inner_current_tracking/1

== system ps_25V_12kA_r/afe_abc_mod1/AFE_control/afe_control/data_to_worspace_module_1/pwr_meter ==
  Bus Creator1 : BusCreator  Inputs=4
  m_pwr_meter : Outport
  wires:
  [u_grid_pu_rms] -> Bus Creator1/2  "u_grid_pu_rms"
  Bus Creator1/1 -> m_pwr_meter/1
  [pwr_act_grid] -> Bus Creator1/3  "pwr_act_grid"
  [pwr_react_grid] -> Bus Creator1/4  "pwr_react_grid"
  [i_grid_pu_rms] -> Bus Creator1/1  "i_grid_pu_rms"

== system ps_25V_12kA_r/afe_abc_mod1/AFE_control/afe_control/data_to_worspace_module_1/sequences_data ==
  Bus Creator1 : BusCreator  Inputs=11
  Demux : Demux  Outputs=3
  m_seq : Outport
  wires:
  Bus Creator1/1 -> m_seq/1
  Demux/3 -> Bus Creator1/3  "i_grid_neg_eta_ref"
  Demux/2 -> Bus Creator1/2  "i_grid_neg_xi_ref"
  Demux/1 -> Bus Creator1/1  "i_grid_pos_eta_ref"
  [v_grid_pos_xi_avg] -> Bus Creator1/4  "v_grid_pos_xi_avg"
  [v_grid_pos_eta_avg] -> Bus Creator1/5  "v_grid_pos_eta_avg"
  [v_grid_neg_xi_avg] -> Bus Creator1/6  "v_grid_neg_xi_avg"
  [v_grid_neg_eta_avg] -> Bus Creator1/7  "v_grid_neg_eta_avg"
  [i_grid_pos_xi_avg] -> Bus Creator1/8  "i_grid_pos_xi_avg"
  [i_grid_pos_eta_avg] -> Bus Creator1/9  "i_grid_pos_eta_avg"
  [i_grid_neg_xi_avg] -> Bus Creator1/10  "i_grid_neg_xi_avg"
  [i_grid_neg_eta_avg] -> Bus Creator1/11  "i_grid_neg_eta_avg"
  [i_grid_seq_ref] -> Demux/1
